simulink model "ElectricVehicleThermalManagementWithHeatPump"  (R2024b)
settings: Solver=VariableStepAuto  StartTime=0.0  StopTime=3600  RelTol=1e-3  AbsTol=1e-3
PreLoadFcn:
  | init_nmpc
InitFcn:
  | init_nmpc
model workspace: external: MATLAB File ElectricVehicleThermalManagementWithHeatPumpParameters.m (data not in the file)
values from neighbouring files (symbols this model uses):
  battery_C1_LUT = [1913.6 12447 30609 ... (first row only)    [ElectricVehicleThermalManagementWithHeatPumpParameters.m]
  battery_capacity_LUT = [280.081 276.25 276.392]    [ElectricVehicleThermalManagementWithHeatPumpParameters.m]
  battery_cell_cp = 795    [ElectricVehicleThermalManagementWithHeatPumpParameters.m]
  battery_cell_mass = 2.5    [ElectricVehicleThermalManagementWithHeatPumpParameters.m]
  battery_Em_LUT = [3.4966 3.5057 3.5148 ... (first row only)    [ElectricVehicleThermalManagementWithHeatPumpParameters.m]
  battery_N_cells = 20    [ElectricVehicleThermalManagementWithHeatPumpParameters.m]
  battery_Qe_init = 0    [ElectricVehicleThermalManagementWithHeatPumpParameters.m]
  battery_R0_LUT = [0.0117 0.0085 0.009 ... (first row only)    [ElectricVehicleThermalManagementWithHeatPumpParameters.m]
  battery_R1_LUT = [0.0109 0.0029 0.0013 ... (first row only)    [ElectricVehicleThermalManagementWithHeatPumpParameters.m]
  battery_SOC_LUT = [0; 0.1; 0.25; 0.5; 0.75; 0.9; 1]    [ElectricVehicleThermalManagementWithHeatPumpParameters.m]
  battery_T_init = -10    [ElectricVehicleThermalManagementWithHeatPumpParameters.m]
  battery_temperature_LUT = [5 20 40]    [ElectricVehicleThermalManagementWithHeatPumpParameters.m]
  cabin_duct_area = 0.04    [ElectricVehicleThermalManagementWithHeatPumpParameters.m]
  cabin_T_init = -10    [ElectricVehicleThermalManagementWithHeatPumpParameters.m]
  chiller_area_primary = 0.43982297150257105    (= 0.439822971503)    [ElectricVehicleThermalManagementWithHeatPumpParameters.m]
  chiller_N_baffles = 3    [ElectricVehicleThermalManagementWithHeatPumpParameters.m]
  chiller_N_tubes = 100    [ElectricVehicleThermalManagementWithHeatPumpParameters.m]
  chiller_tube_D = 0.0035    [ElectricVehicleThermalManagementWithHeatPumpParameters.m]
  chiller_tube_L = 0.4    [ElectricVehicleThermalManagementWithHeatPumpParameters.m]
  chiller_wall_conductivity = 240    [ElectricVehicleThermalManagementWithHeatPumpParameters.m]
  chiller_wall_thickness = 0.0001    [ElectricVehicleThermalManagementWithHeatPumpParameters.m]
  cond_evap_air_area_flow = 0.3906    [ElectricVehicleThermalManagementWithHeatPumpParameters.m]
  cond_evap_air_area_primary = 1.4834999999999998    (= 1.4835)    [ElectricVehicleThermalManagementWithHeatPumpParameters.m]
  cond_evap_W = 0.015    [ElectricVehicleThermalManagementWithHeatPumpParameters.m]
  cond_evap_wall_conductivity = 240    [ElectricVehicleThermalManagementWithHeatPumpParameters.m]
  cond_evap_wall_thickness = 0.0001    [ElectricVehicleThermalManagementWithHeatPumpParameters.m]
  coolant_channel_D = 0.0092    [ElectricVehicleThermalManagementWithHeatPumpParameters.m]
  coolant_pipe_D = 0.019    [ElectricVehicleThermalManagementWithHeatPumpParameters.m]
  coolant_T_init = -10    [ElectricVehicleThermalManagementWithHeatPumpParameters.m]
  coolant_tank_area = 0.0121    [ElectricVehicleThermalManagementWithHeatPumpParameters.m]
  coolant_tank_volume = 1.25    [ElectricVehicleThermalManagementWithHeatPumpParameters.m]
  coolant_valve_D_ratio_max = 0.95    [ElectricVehicleThermalManagementWithHeatPumpParameters.m]
  coolant_valve_D_ratio_min = 0.001    [ElectricVehicleThermalManagementWithHeatPumpParameters.m]
  coolant_valve_displacement = 0.0063    [ElectricVehicleThermalManagementWithHeatPumpParameters.m]
  coolant_valve_S_max = 0.0053    [ElectricVehicleThermalManagementWithHeatPumpParameters.m]
  evaporator_air_area_flow = 0.12    [ElectricVehicleThermalManagementWithHeatPumpParameters.m]
  evaporator_air_area_primary = 0.4323    [ElectricVehicleThermalManagementWithHeatPumpParameters.m]
  evaporator_W = 0.015    [ElectricVehicleThermalManagementWithHeatPumpParameters.m]
  evaporator_wall_conductivity = 240    [ElectricVehicleThermalManagementWithHeatPumpParameters.m]
  evaporator_wall_thickness = 0.0001    [ElectricVehicleThermalManagementWithHeatPumpParameters.m]
  expansion_valve_D_ratio_max = 0.9    [ElectricVehicleThermalManagementWithHeatPumpParameters.m]
  hex_area_primary = 0.070371675440411369    (= 0.0703716754404)    [ElectricVehicleThermalManagementWithHeatPumpParameters.m]
  hex_N_tubes = 64    [ElectricVehicleThermalManagementWithHeatPumpParameters.m]
  hex_tube_D = 0.0035    [ElectricVehicleThermalManagementWithHeatPumpParameters.m]
  hex_wall_conductivity = 240    [ElectricVehicleThermalManagementWithHeatPumpParameters.m]
  hex_wall_thickness = 0.0001    [ElectricVehicleThermalManagementWithHeatPumpParameters.m]
  inner_cond_air_area_flow = 0.1953    [ElectricVehicleThermalManagementWithHeatPumpParameters.m]
  inner_cond_air_area_primary = 0.99520000000000008    (= 0.9952)    [ElectricVehicleThermalManagementWithHeatPumpParameters.m]
  inner_cond_W = 0.02    [ElectricVehicleThermalManagementWithHeatPumpParameters.m]
  inner_cond_wall_conductivity = 240    [ElectricVehicleThermalManagementWithHeatPumpParameters.m]
  inner_cond_wall_thickness = 0.0001    [ElectricVehicleThermalManagementWithHeatPumpParameters.m]
  pump_speed_max = 1000    [ElectricVehicleThermalManagementWithHeatPumpParameters.m]
  radiator_air_area_flow = 0.097499999999999989    (= 0.0975)    [ElectricVehicleThermalManagementWithHeatPumpParameters.m]
  radiator_air_area_primary = 0.43687499999999996    (= 0.436875)    [ElectricVehicleThermalManagementWithHeatPumpParameters.m]
  radiator_W = 0.015    [ElectricVehicleThermalManagementWithHeatPumpParameters.m]
  radiator_wall_conductivity = 240    [ElectricVehicleThermalManagementWithHeatPumpParameters.m]
  radiator_wall_thickness = 0.0001    [ElectricVehicleThermalManagementWithHeatPumpParameters.m]
  refrigerant_p_init = 0.2    [ElectricVehicleThermalManagementWithHeatPumpParameters.m]
  refrigerant_pipe_D = 0.01    [ElectricVehicleThermalManagementWithHeatPumpParameters.m]
  refrigerant_valve_D_ratio_max = 0.95    [ElectricVehicleThermalManagementWithHeatPumpParameters.m]
  refrigerant_valve_displacement = 0.005    [ElectricVehicleThermalManagementWithHeatPumpParameters.m]
libraries: fl_lib x227, nesl_utility x162, SimscapeFluids_lib x30, LiBatteryElements_lib x16, slpidlib x3, SignalEditorBlockLib x1
(part 5 of 13)

== system ElectricVehicleThermalManagementWithHeatPump/Evaporator ==
  Evaporator : SimscapeFluids_lib/Heat Exchangers/Two-Phase Fluid - Moist Air/Condenser Evaporator (2P-MA)  flow_arrangement=fluids.heat_exchangers.enum.FlowArrangement2PMA.Cross  cross_flow_arrangement=fluids.heat_exchangers.enum.CrossFlowArrangement2PMA.UnmixedUnmixed  R_wall=evaporator_wall_thickness / evaporator_air_area_primary / evaporator_wall_conductivity K/W  area_A1=pi * refrigerant_pipe_D^2 / 4 m^2  area_B1=pi * refrigerant_pipe_D^2 / 4 m^2  area_A2=cabin_duct_area m^2  area_B2=cabin_duct_area m^2  tube_num_2P=evaporator_N_tubes  tube_length_2P=evaporator_L m  tube_cross_section_2P=fluids.heat_exchangers.enum.TubeCrossSection.Rectangular  tube_diameter_2P=0.1 m  tube_width_2P=evaporator_W m  tube_height_2P=evaporator_tube_H m  tube_inner_diameter_2P=0.05 m  tube_outer_diameter_2P=0.1 m  tube_flow_area_2P=0.01 m^2  tube_wetted_perimeter_2P=0.4 m  tube_heat_perimeter_2P=0.4 m  tube_pressure_loss_spec_2P=fluids.heat_exchangers.enum.TubePressureLossSpec2P.Haaland  tube_loss_coeff_2P=10  tube_local_pressure_loss_spec_2P=fluids.heat_exchangers.enum.LocalLossSpec.AggregateLength  tube_length_add_2P=evaporator_tube_Leq m  tube_local_loss_coefficient_2P=0.1  tube_roughness_pressure_2P=15e-6 m  tube_Re_lam_pressure_2P=2000  tube_Re_tur_pressure_2P=4000  tube_shape_factor_generic_2P=64  tube_heat_coeff_spec_2P=fluids.heat_exchangers.enum.TubeHeatCoeffSpec2P.GneilinskiCavalliniZecchin  tube_colburn_coeff_liq_2P=[.023, .8, .33]  tube_colburn_coeff_mix_2P=[.05, .8, .33]  tube_colburn_coeff_vap_2P=[.023, .8, .33]  tube_roughness_heat_2P=15e-6 m  tube_Re_lam_heat_2P=2000  tube_Re_tur_heat_2P=4000  tube_Nu_lam_generic_2P=3.66  fouling_factor_2P=0.1 m^2*K/kW  fin_area_2P=evaporator_tube_area_webs m^2  fin_efficiency_2P=0.6  energy_spec_2P=foundation.enum.energy_spec.void_fraction  p_init_2P=refrigerant_p_init MPa  T_init_2P=293.15 K  x_init_2P=0.5  alpha_init_2P=refrigerant_alpha_init  h_init_2P=1500 kJ/kg  u_init_2P=1500 kJ/kg  flow_geometry_MA=fluids.heat_exchangers.enum.FlowGeometryMA.Generic  tube_num_MA=1  tube_length_MA=5 m  tube_cross_section_MA=fluids.heat_exchangers.enum.TubeCrossSection.Circular  tube_diameter_MA=0.1 m  tube_width_MA=0.1 m  tube_height_MA=0.1 m  tube_inner_diameter_MA=0.05 m  tube_outer_diameter_MA=0.1 m  tube_flow_area_MA=0.01 m^2  tube_wetted_perimeter_MA=0.4 m  tube_heat_perimeter_MA=0.4 m  tube_pressure_loss_spec_MA=fluids.heat_exchangers.enum.TubePressureLossSpec.Haaland  tube_loss_coeff_MA=10  tube_local_pressure_loss_spec_MA=fluids.heat_exchangers.enum.LocalLossSpec.AggregateLength  tube_length_add_MA=0.1 m  tube_local_loss_coefficient_MA=0.1  tube_roughness_pressure_MA=15e-6 m  tube_Re_lam_pressure_MA=2000  tube_Re_tur_pressure_MA=4000  tube_shape_factor_generic_MA=64  tube_heat_coeff_spec_MA=fluids.heat_exchangers.enum.TubeHeatCoeffSpec.Gneilinski  tube_colburn_coeff_MA=[.023, .8, .33]  tube_roughness_heat_MA=15e-6 m  tube_Re_lam_heat_MA=2000  tube_Re_tur_heat_MA=4000  tube_Nu_lam_generic_MA=3.66  bank_arrangement_MA=fluids.heat_exchangers.enum.BankArrangement.Inline  bank_num_rows_MA=5  bank_tubes_per_row_MA=5  bank_width_MA=1 m  bank_tube_diameter_MA=0.05 m  bank_longitudinal_pitch_MA=0.15 m  bank_transverse_pitch_MA=0.15 m  bank_pressure_loss_spec_MA=fluids.heat_exchangers.enum.BankPressureLossSpec.Martin  bank_euler_MA=10  bank_heat_coeff_spec_MA=fluids.heat_exchangers.enum.BankHeatCoeffSpec.Martin  bank_colburn_coeff_MA=[.27, .63, .36]  generic_flow_area_MA=evaporator_air_area_flow m^2  generic_heat_area_MA=evaporator_air_area_primary m^2  generic_volume_MA=evaporator_air_area_flow * evaporator_W m^3  generic_loss_coeff_MA=10  generic_colburn_coeff_MA=[0.27, 0.63, 0.36]  fouling_factor_MA=0.1 m^2*K/kW  fin_area_MA=evaporator_air_area_fins m^2  fin_efficiency_MA=0.7  p_init_MA=cabin_p_init MPa  T_init_MA=cabin_T_init degC  humidity_spec_MA=foundation.enum.HumiditySpec.RelativeHumidity  RH_init_MA=cabin_RH_init  x_w_init_MA=0.01  y_w_init_MA=0.01  HR_init_MA=0.01  Tw_init_MA=287 K  trace_gas_spec_MA=foundation.enum.trace_gas_spec.mole_fraction  x_g_init_MA=0.001  y_g_init_MA=cabin_CO2_init  r_d_init_MA=0  RH_ws_MA=1  time_constant_cond_MA=1e-3 s  time_constant_evap_MA=1e-3 s  fraction_entrained_MA=1
      settings: InternalSimscapePortConfiguration="{\"Bottom\":[],\"Left\":[{\"id\":\"A1\",\"label\":\"A1\",\"type\":\"foundation.two_phase_fluid.two_phase_fluid\"},{\"id\":\"Z\",\"label\":\"Z\",\"type\":\"output\"},{\"id\":\"B1\",\"label\":\"B1\",\"type\":\"foundation.two_phase_fluid.two_phase_fluid\"}],\"Right\":[{\"id\":\"A2\",\"label\":\"A2\",\"type\":\"foundation.moist_air.moist_air\"},{\"id\":\"W\",\"label\":\"W\",\"type\":\"output\"},{\"id\":\"B2\",\"label\":\"B2\",\"type\":\"foundation.moist_air.moist_air\"}],\"Top\":[]}"
  Flow Resistance (2P) : fl_lib/Two-Phase Fluid/Elements/Flow Resistance (2P)  delta_p_nominal=1e-4 MPa  mdot_nominal=0.01 kg/s  v_nominal=0 m^3/kg  area=pi * refrigerant_pipe_D^2 / 4 m^2  laminar_fraction=1e-3
      settings: InternalSimscapePortConfiguration="{\"Bottom\":[],\"Left\":[{\"id\":\"A\",\"label\":\"A\",\"type\":\"foundation.two_phase_fluid.two_phase_fluid\"}],\"Right\":[{\"id\":\"B\",\"label\":\"B\",\"type\":\"foundation.two_phase_fluid.two_phase_fluid\"}],\"Top\":[]}"
  PS-Simulink Converter{,1..3} (4 alike) : nesl_utility/PS-Simulink Converter  PhysicalDomain=network_engine_domain  SubClassName=ps_output  LeftPortType=input  RightPortType=output  PseudoPeriodic=off  Frequencies=[]  VectorFormat=inherit  Unit=inherit  AffineConversion=off
  Pressure & Temperature Sensor (MA) : fl_lib/Moist Air/Sensors/Pressure & Temperature Sensor (MA)  reference=foundation.enum.MeasurementReference.absolute  pressure=true  pressure_spec=foundation.enum.PressureMeasementSpec.Absolute  temperature=true
      settings: InternalSimscapePortConfiguration="{\"Bottom\":[{\"id\":\"T\",\"label\":\"T\",\"type\":\"output\"}],\"Left\":[{\"id\":\"A\",\"label\":\"A\",\"type\":\"foundation.moist_air.moist_air\"}],\"Right\":[{\"id\":\"Pa\",\"label\":\"Pa\",\"type\":\"output\"}],\"Top\":[]}"
  Pressure & Temperature Sensor (MA)1 : fl_lib/Moist Air/Sensors/Pressure & Temperature Sensor (MA)  reference=foundation.enum.MeasurementReference.absolute  pressure=true  pressure_spec=foundation.enum.PressureMeasementSpec.Absolute  temperature=true
      settings: InternalSimscapePortConfiguration="{\"Bottom\":[{\"id\":\"T\",\"label\":\"T\",\"type\":\"output\"}],\"Left\":[{\"id\":\"A\",\"label\":\"A\",\"type\":\"foundation.moist_air.moist_air\"}],\"Right\":[{\"id\":\"Pa\",\"label\":\"Pa\",\"type\":\"output\"}],\"Top\":[]}"
  SR7 : Subsystem
  SR8 : Subsystem
  Scope : Scope
  To Workspace : ToWorkspace  VariableName=airEvapPressure_out  SampleTime=-1
  To Workspace1 : ToWorkspace  VariableName=airEvapTemp_out  SampleTime=-1
  To Workspace2 : ToWorkspace  VariableName=airEvapPressure_in  SampleTime=-1
  To Workspace3 : ToWorkspace  VariableName=airEvapTemp_in  SampleTime=-1
  A : PMIOPort  Side=Left
  D : PMIOPort  Port=2  Side=Left
  B : PMIOPort  Port=3  Side=Right
  C : PMIOPort  Port=4  Side=Right
  wires:
  PS-Simulink Converter/1 -> To Workspace/1
  PS-Simulink Converter3/1 -> Scope/1, To Workspace1/1
  PS-Simulink Converter1/1 -> To Workspace2/1
  PS-Simulink Converter2/1 -> To Workspace3/1
  connections:
  SR8/LConn1 -- Evaporator/LConn3
  SR7/RConn1 -- Evaporator/LConn1
  SR8/RConn1 -- Flow Resistance (2P)/LConn1
  Evaporator/RConn3 -- Pressure & Temperature Sensor (MA)1/LConn1 -- C/RConn1
  Flow Resistance (2P)/RConn1 -- B/RConn1
  Evaporator/RConn1 -- D/RConn1 -- Pressure & Temperature Sensor (MA)/LConn1
  SR7/LConn1 -- A/RConn1
  PS-Simulink Converter/LConn1 -- Pressure & Temperature Sensor (MA)/RConn1
  PS-Simulink Converter1/LConn1 -- Pressure & Temperature Sensor (MA)1/RConn1
  PS-Simulink Converter2/LConn1 -- Pressure & Temperature Sensor (MA)1/RConn2
  PS-Simulink Converter3/LConn1 -- Pressure & Temperature Sensor (MA)/RConn2

== system ElectricVehicleThermalManagementWithHeatPump/Evaporator Expansion Valve ==
  Evaporator Expansion Valve : SimscapeFluids_lib/Two-Phase Fluid/Valves & Orifices/Orifice (2P)  orifice_type=foundation.enum.constant_variable.variable  constant_liquid_orifice_parameterization=fluids.two_phase_fluid.valves_orifices.enum.LiquidConstantOrificeParameterization.Area  variable_liquid_orifice_parameterization=fluids.two_phase_fluid.valves_orifices.enum.LiquidOrificeParameterization.LinearArea  mdot_nominal_constant=0.1 kg/s  delta_p_nominal_constant=0.001 MPa  orifice_area_constant=1e-4 m^2  S_min=0 m  del_S=refrigerant_valve_displacement m  open_orientation=fluids.two_phase_fluid.valves_orifices.enum.OrificeOrientation.Positive  mdot_nominal_max=0.1 kg/s  delta_p_nominal_max=0.001 MPa  orifice_area_max=pi * (expansion_valve_D_ratio_max*refrigerant_pipe_D)^2 / 4 m^2  S_TLU=[0, .002, .004, .007, .017] m  orifice_area_TLU=[1e-10, 2e-05, 4e-05, 6e-05, 8e-05, .0001] m^2  energy_spec=foundation.enum.energy_spec.temperature  p_inlet=0.101325 MPa  T_inlet=293.15 K  x_inlet=0  alpha_inlet=0  h_inlet=400 kJ/kg  u_inlet=400 kJ/kg  Cd=0.7  pressure_recovery=true  leakage_fraction=1e-6  smoothing_factor=0.01  B_lam=0.999  tau_x=0.1 s  area=pi * refrigerant_pipe_D^2 / 4 m^2  vapor_orifice_parameterization=fluids.two_phase_fluid.valves_orifices.enum.VaporOrificeParameterization.Cv  opening_characteristic=fluids.two_phase_fluid.valves_orifices.enum.OpeningCharacteristics.Linear  Cv_constant=4  Cv_max=4  S_Cv_TLU=[0, .003, .006, .009, .012, .015] m  Cv_TLU=[1e-06, .8, 1.6, 2.4, 3.2, 4]  xT_Cv=0.7  Kv_constant=3.6  Kv_max=3.6  S_Kv_TLU=[0, .003, .006, .009, .012, .015] m  Kv_TLU=[1e-06, .72, 1.44, 2.16, 2.88, 3.6]  xT_Kv=0.7  S_orifice_area_TLU=[0, .003, .006, .009, .012, .015] m
      settings: InternalSimscapePortConfiguration="{\"Bottom\":[],\"Left\":[{\"id\":\"A\",\"label\":\"A\",\"type\":\"foundation.two_phase_fluid.two_phase_fluid\"},{\"id\":\"S\",\"label\":\"S\",\"type\":\"input\"}],\"Right\":[{\"id\":\"B\",\"label\":\"B\",\"type\":\"foundation.two_phase_fluid.two_phase_fluid\"}],\"Top\":[]}"
  Max Valve Displacement [m] : Gain  Gain=refrigerant_valve_displacement
  Simulink-PS Converter : nesl_utility/Simulink-PS Converter  PhysicalDomain=network_engine_domain  SubClassName=ps_input  LeftPortType=input  RightPortType=output  PseudoPeriodic=off  Frequencies=[]  NoiseDistribution=none  NoiseParameters=[]  Unit=m  AffineConversion=off  FilteringAndDerivatives=provide  SimscapeFilterOrder=1  InputFilterTimeConstant=0.001  UdotUserProvided=0
  Transfer Fcn : TransferFcn  Denominator=[1 1]
  A : PMIOPort  Side=Left
  B : PMIOPort  Port=2  Side=Right
  wires:
  Transfer Fcn/1 -> Max Valve Displacement [m]/1
  [cmd_exv_evap] -> Transfer Fcn/1
  Max Valve Displacement [m]/1 -> Simulink-PS Converter/1
  connections:
  Evaporator Expansion Valve/LConn2 -- Simulink-PS Converter/RConn1
  Evaporator Expansion Valve/LConn1 -- A/RConn1
  Evaporator Expansion Valve/RConn1 -- B/RConn1

== system ElectricVehicleThermalManagementWithHeatPump/Heat Exchanger ==
  Flow Rate Sensor (TL) : fl_lib/Thermal Liquid/Sensors/Flow Rate Sensor (TL)  mass_flow_measure=true  volumetric_flow_measure=false  energy_flow_measure=true
      settings: InternalSimscapePortConfiguration="{\"Bottom\":[{\"id\":\"PHI\",\"label\":\"φ\",\"type\":\"output\"}],\"Left\":[{\"id\":\"A\",\"label\":\"A\",\"type\":\"foundation.thermal_liquid.thermal_liquid\"}],\"Right\":[{\"id\":\"B\",\"label\":\"B\",\"type\":\"foundation.thermal_liquid.thermal_liquid\"},{\"id\":\"M\",\"label\":\"M\",\"type\":\"output\"}],\"Top\":[]}"
  Heat Exchanger : SimscapeFluids_lib/Heat Exchangers/Two-Phase Fluid - Thermal Liquid/Condenser Evaporator (TL-2P)  flow_arrangement=fluids.heat_exchangers.enum.FlowArrangementTL2P.Cross  cross_flow_arrangement=fluids.heat_exchangers.enum.CrossFlowArrangementTL2P.UnmixedMixed  R_wall=hex_wall_thickness / hex_area_primary / hex_wall_conductivity K/W  area_A1=pi * coolant_pipe_D^2 / 4 m^2  area_B1=pi * coolant_pipe_D^2 / 4 m^2  area_A2=pi * refrigerant_pipe_D^2 / 4 m^2  area_B2=pi * refrigerant_pipe_D^2 / 4 m^2  flow_geometry_TL=fluids.heat_exchangers.enum.FlowGeometryTL.AcrossTubeBank  tube_num_TL=1  tube_length_TL=5 m  tube_cross_section_TL=fluids.heat_exchangers.enum.TubeCrossSection.Circular  tube_diameter_TL=0.1 m  tube_width_TL=0.1 m  tube_height_TL=0.1 m  tube_inner_diameter_TL=0.05 m  tube_outer_diameter_TL=0.1 m  tube_flow_area_TL=0.01 m^2  tube_wetted_perimeter_TL=0.4 m  tube_heat_perimeter_TL=0.4 m  tube_pressure_loss_spec_TL=fluids.heat_exchangers.enum.TubePressureLossSpec.Haaland  tube_loss_coeff_TL=10  tube_local_pressure_loss_spec_TL=fluids.heat_exchangers.enum.LocalLossSpec.AggregateLength  tube_length_add_TL=0.1 m  tube_local_loss_coefficient_TL=0.1  tube_roughness_pressure_TL=15e-6 m  tube_Re_lam_pressure_TL=2000  tube_Re_tur_pressure_TL=4000  tube_shape_factor_generic_TL=64  tube_heat_coeff_spec_TL=fluids.heat_exchangers.enum.TubeHeatCoeffSpec.Gneilinski  tube_colburn_coeff_TL=[.023, .8, .33]  tube_roughness_heat_TL=15e-6 m  tube_Re_lam_heat_TL=2000  tube_Re_tur_heat_TL=4000  tube_Nu_lam_generic_TL=3.66  bank_arrangement_TL=fluids.heat_exchangers.enum.BankArrangement.Staggered  bank_num_rows_TL=sqrt(hex_N_tubes)  bank_tubes_per_row_TL=sqrt(hex_N_tubes)  bank_width_TL=hex_tube_L m  bank_tube_diameter_TL=hex_tube_D m  bank_longitudinal_pitch_TL=2 * hex_tube_D m  bank_transverse_pitch_TL=2 * hex_tube_D m  bank_pressure_loss_spec_TL=fluids.heat_exchangers.enum.BankPressureLossSpec.Martin  bank_euler_TL=10  bank_heat_coeff_spec_TL=fluids.heat_exchangers.enum.BankHeatCoeffSpec.Martin  bank_colburn_coeff_TL=[.27, .63, .36]  generic_flow_area_TL=0.01 m^2  generic_heat_area_TL=2 m^2  generic_volume_TL=0.05 m^3  generic_loss_coeff_TL=10  generic_colburn_coeff_TL=[.023, .8, .33]  fouling_factor_TL=0.1 m^2*K/kW  fin_area_TL=0 m^2  fin_efficiency_TL=0  p_init_TL=coolant_p_init MPa  T_init_TL=coolant_T_init degC  tube_num_2P=hex_N_tubes  tube_length_2P=hex_tube_L m  tube_cross_section_2P=fluids.heat_exchangers.enum.TubeCrossSection.Circular  tube_diameter_2P=hex_tube_D m  tube_width_2P=0.1 m  tube_height_2P=0.1 m  tube_inner_diameter_2P=0.05 m  tube_outer_diameter_2P=0.1 m  tube_flow_area_2P=0.01 m^2  tube_wetted_perimeter_2P=0.4 m  tube_heat_perimeter_2P=0.4 m  tube_pressure_loss_spec_2P=fluids.heat_exchangers.enum.TubePressureLossSpec2P.Haaland  tube_loss_coeff_2P=10  tube_local_pressure_loss_spec_2P=fluids.heat_exchangers.enum.LocalLossSpec.AggregateLength  tube_length_add_2P=hex_tube_Leq m  tube_local_loss_coefficient_2P=0.1  tube_roughness_pressure_2P=15e-6 m  tube_Re_lam_pressure_2P=2000  tube_Re_tur_pressure_2P=4000  tube_shape_factor_generic_2P=64  tube_heat_coeff_spec_2P=fluids.heat_exchangers.enum.TubeHeatCoeffSpec2P.GneilinskiCavalliniZecchin  tube_colburn_coeff_liq_2P=[.023, .8, .33]  tube_colburn_coeff_mix_2P=[.05, .8, .33]  tube_colburn_coeff_vap_2P=[.023, .8, .33]  tube_roughness_heat_2P=15e-6 m  tube_Re_lam_heat_2P=2000  tube_Re_tur_heat_2P=4000  tube_Nu_lam_generic_2P=3.66  fouling_factor_2P=0.1 m^2*K/kW  fin_area_2P=0 m^2  fin_efficiency_2P=0  energy_spec_2P=foundation.enum.energy_spec.void_fraction  p_init_2P=refrigerant_p_init MPa  T_init_2P=293.15 K  x_init_2P=0.5  alpha_init_2P=refrigerant_alpha_init  h_init_2P=1500 kJ/kg  u_init_2P=1500 kJ/kg
      settings: InternalSimscapePortConfiguration="{\"Bottom\":[],\"Left\":[{\"id\":\"A1\",\"label\":\"A1\",\"type\":\"foundation.thermal_liquid.thermal_liquid\"},{\"id\":\"B1\",\"label\":\"B1\",\"type\":\"foundation.thermal_liquid.thermal_liquid\"}],\"Right\":[{\"id\":\"A2\",\"label\":\"A2\",\"type\":\"foundation.two_phase_fluid.two_phase_fluid\"},{\"id\":\"B2\",\"label\":\"B2\",\"type\":\"foundation.two_phase_fluid.two_phase_fluid\"}],\"Top\":[{\"id\":\"Z\",\"label\":\"Z\",\"type\":\"output\"}]}"
  PS-Simulink Converter : nesl_utility/PS-Simulink Converter  PhysicalDomain=network_engine_domain  SubClassName=ps_output  LeftPortType=input  RightPortType=output  PseudoPeriodic=off  Frequencies=[]  VectorFormat=inherit  Unit=inherit  AffineConversion=off
  PS-Simulink Converter1 : nesl_utility/PS-Simulink Converter  PhysicalDomain=network_engine_domain  SubClassName=ps_output  LeftPortType=input  RightPortType=output  PseudoPeriodic=off  Frequencies=[]  VectorFormat=inherit  Unit=inherit  AffineConversion=off
  PS-Simulink Converter2 : nesl_utility/PS-Simulink Converter  PhysicalDomain=network_engine_domain  SubClassName=ps_output  LeftPortType=input  RightPortType=output  PseudoPeriodic=off  Frequencies=[]  VectorFormat=inherit  Unit=inherit  AffineConversion=off
  Pressure & Temperature Sensor (TL) : fl_lib/Thermal Liquid/Sensors/Pressure & Temperature Sensor (TL)  reference=foundation.enum.MeasurementReference.absolute  pressure=false  pressure_spec=foundation.enum.PressureMeasementSpec.Absolute  temperature=true
      settings: InternalSimscapePortConfiguration="{\"Bottom\":[{\"id\":\"T\",\"label\":\"T\",\"type\":\"output\"}],\"Left\":[{\"id\":\"A\",\"label\":\"A\",\"type\":\"foundation.thermal_liquid.thermal_liquid\"}],\"Right\":[],\"Top\":[]}"
  Pressure & Temperature Sensor (TL)1 : fl_lib/Thermal Liquid/Sensors/Pressure & Temperature Sensor (TL)  reference=foundation.enum.MeasurementReference.absolute  pressure=false  pressure_spec=foundation.enum.PressureMeasementSpec.Absolute  temperature=true
      settings: InternalSimscapePortConfiguration="{\"Bottom\":[{\"id\":\"T\",\"label\":\"T\",\"type\":\"output\"}],\"Left\":[{\"id\":\"A\",\"label\":\"A\",\"type\":\"foundation.thermal_liquid.thermal_liquid\"}],\"Right\":[],\"Top\":[]}"
  SR5 : Subsystem
  SR6 : Subsystem
  Scope : Scope
  Scope1 : Scope
  Scope2 : Scope
  To Workspace : ToWorkspace  VariableName=heatExchangerCoolantT_outK  SampleTime=-1
  To Workspace1 : ToWorkspace  VariableName=heatExchangerCoolantT_inK  SampleTime=-1
  To Workspace2 : ToWorkspace  VariableName=mf_htxClnt  SampleTime=-1
  D : PMIOPort  Side=Left
  A : PMIOPort  Port=2  Side=Left
  C : PMIOPort  Port=3  Side=Right
  B : PMIOPort  Port=4  Side=Right
  wires:
  PS-Simulink Converter/1 -> To Workspace/1, Scope/1
  PS-Simulink Converter1/1 -> Scope1/1, To Workspace1/1
  PS-Simulink Converter2/1 -> To Workspace2/1, Scope2/1
  connections:
  Heat Exchanger/RConn2 -- SR6/LConn1
  SR6/RConn1 -- B/RConn1
  Heat Exchanger/RConn1 -- SR5/RConn1
  SR5/LConn1 -- A/RConn1
  C/RConn1 -- Pressure & Temperature Sensor (TL)1/LConn1 -- Heat Exchanger/LConn2
  Pressure & Temperature Sensor (TL)/LConn1 -- D/RConn1 -- Flow Rate Sensor (TL)/RConn1
  PS-Simulink Converter/LConn1 -- Pressure & Temperature Sensor (TL)/RConn1
  PS-Simulink Converter1/LConn1 -- Pressure & Temperature Sensor (TL)1/RConn1
  PS-Simulink Converter2/LConn1 -- Flow Rate Sensor (TL)/RConn2
  Flow Rate Sensor (TL)/LConn1 -- Heat Exchanger/LConn1

== system ElectricVehicleThermalManagementWithHeatPump/Heat Pump Expansion Valve ==
  Heat Pump Expansion Valve : SimscapeFluids_lib/Two-Phase Fluid/Valves & Orifices/Orifice (2P)  orifice_type=foundation.enum.constant_variable.variable  constant_liquid_orifice_parameterization=fluids.two_phase_fluid.valves_orifices.enum.LiquidConstantOrificeParameterization.Area  variable_liquid_orifice_parameterization=fluids.two_phase_fluid.valves_orifices.enum.LiquidOrificeParameterization.LinearArea  mdot_nominal_constant=0.1 kg/s  delta_p_nominal_constant=0.001 MPa  orifice_area_constant=1e-4 m^2  S_min=0 m  del_S=refrigerant_valve_displacement m  open_orientation=fluids.two_phase_fluid.valves_orifices.enum.OrificeOrientation.Positive  mdot_nominal_max=0.1 kg/s  delta_p_nominal_max=0.001 MPa  orifice_area_max=pi * (expansion_valve_D_ratio_max*refrigerant_pipe_D)^2 / 4 m^2  S_TLU=[0, .002, .004, .007, .017] m  orifice_area_TLU=[1e-10, 2e-05, 4e-05, 6e-05, 8e-05, .0001] m^2  energy_spec=foundation.enum.energy_spec.temperature  p_inlet=0.101325 MPa  T_inlet=293.15 K  x_inlet=0  alpha_inlet=0  h_inlet=400 kJ/kg  u_inlet=400 kJ/kg  Cd=0.7  pressure_recovery=true  leakage_fraction=1e-6  smoothing_factor=0.01  B_lam=0.999  tau_x=0.1 s  area=pi * refrigerant_pipe_D^2 / 4 m^2  vapor_orifice_parameterization=fluids.two_phase_fluid.valves_orifices.enum.VaporOrificeParameterization.Cv  opening_characteristic=fluids.two_phase_fluid.valves_orifices.enum.OpeningCharacteristics.Linear  Cv_constant=4  Cv_max=4  S_Cv_TLU=[0, .003, .006, .009, .012, .015] m  Cv_TLU=[1e-06, .8, 1.6, 2.4, 3.2, 4]  xT_Cv=0.7  Kv_constant=3.6  Kv_max=3.6  S_Kv_TLU=[0, .003, .006, .009, .012, .015] m  Kv_TLU=[1e-06, .72, 1.44, 2.16, 2.88, 3.6]  xT_Kv=0.7  S_orifice_area_TLU=[0, .003, .006, .009, .012, .015] m
      settings: InternalSimscapePortConfiguration="{\"Bottom\":[],\"Left\":[{\"id\":\"A\",\"label\":\"A\",\"type\":\"foundation.two_phase_fluid.two_phase_fluid\"},{\"id\":\"S\",\"label\":\"S\",\"type\":\"input\"}],\"Right\":[{\"id\":\"B\",\"label\":\"B\",\"type\":\"foundation.two_phase_fluid.two_phase_fluid\"}],\"Top\":[]}"
  Max Valve Displacement [m] : Gain  Gain=refrigerant_valve_displacement
  PS-Simulink Converter : nesl_utility/PS-Simulink Converter  PhysicalDomain=network_engine_domain  SubClassName=ps_output  LeftPortType=input  RightPortType=output  PseudoPeriodic=off  Frequencies=[]  VectorFormat=inherit  Unit=inherit  AffineConversion=off
  PS-Simulink Converter1 : nesl_utility/PS-Simulink Converter  PhysicalDomain=network_engine_domain  SubClassName=ps_output  LeftPortType=input  RightPortType=output  PseudoPeriodic=off  Frequencies=[]  VectorFormat=inherit  Unit=inherit  AffineConversion=off
  "Pressure, Temperature & Internal Energy Sensor (2P)" : fl_lib/Two-Phase Fluid/Sensors/Pressure, Temperature & Internal Energy Sensor (2P)  reference=foundation.enum.MeasurementReference.absolute  pressure=true  pressure_spec=foundation.enum.PressureMeasementSpec.Absolute  temperature=false  internal_energy=false
      settings: InternalSimscapePortConfiguration="{\"Bottom\":[],\"Left\":[{\"id\":\"A\",\"label\":\"A\",\"type\":\"foundation.two_phase_fluid.two_phase_fluid\"}],\"Right\":[{\"id\":\"Pa\",\"label\":\"Pa\",\"type\":\"output\"}],\"Top\":[]}"
  "Pressure, Temperature & Internal Energy Sensor (2P)1" : fl_lib/Two-Phase Fluid/Sensors/Pressure, Temperature & Internal Energy Sensor (2P)  reference=foundation.enum.MeasurementReference.absolute  pressure=true  pressure_spec=foundation.enum.PressureMeasementSpec.Absolute  temperature=false  internal_energy=false
      settings: InternalSimscapePortConfiguration="{\"Bottom\":[],\"Left\":[{\"id\":\"A\",\"label\":\"A\",\"type\":\"foundation.two_phase_fluid.two_phase_fluid\"}],\"Right\":[{\"id\":\"Pa\",\"label\":\"Pa\",\"type\":\"output\"}],\"Top\":[]}"
  Scope : Scope
  Simulink-PS Converter : nesl_utility/Simulink-PS Converter  PhysicalDomain=network_engine_domain  SubClassName=ps_input  LeftPortType=input  RightPortType=output  PseudoPeriodic=off  Frequencies=[]  NoiseDistribution=none  NoiseParameters=[]  Unit=m  AffineConversion=off  FilteringAndDerivatives=provide  SimscapeFilterOrder=1  InputFilterTimeConstant=0.001  UdotUserProvided=0
  To Workspace : ToWorkspace  VariableName=EXVRefPress_inMpa  SampleTime=-1
  To Workspace1 : ToWorkspace  VariableName=EXVRefPress_outMpa  SampleTime=-1
  Transfer Fcn : TransferFcn  Denominator=[1 1]
  B : PMIOPort  Side=Left
  A : PMIOPort  Port=2  Side=Right
  wires:
  Max Valve Displacement [m]/1 -> Scope/1, Simulink-PS Converter/1
  [cmd_exv_heatpump] -> Transfer Fcn/1
  Transfer Fcn/1 -> Max Valve Displacement [m]/1
  PS-Simulink Converter/1 -> To Workspace/1
  PS-Simulink Converter1/1 -> To Workspace1/1
  connections:
  Heat Pump Expansion Valve/RConn1 -- "Pressure, Temperature & Internal Energy Sensor (2P)1"/LConn1 -- B/RConn1
  Heat Pump Expansion Valve/LConn1 -- "Pressure, Temperature & Internal Energy Sensor (2P)"/LConn1 -- A/RConn1
  Heat Pump Expansion Valve/LConn2 -- Simulink-PS Converter/RConn1
  PS-Simulink Converter/LConn1 -- "Pressure, Temperature & Internal Energy Sensor (2P)"/RConn1
  PS-Simulink Converter1/LConn1 -- "Pressure, Temperature & Internal Energy Sensor (2P)1"/RConn1

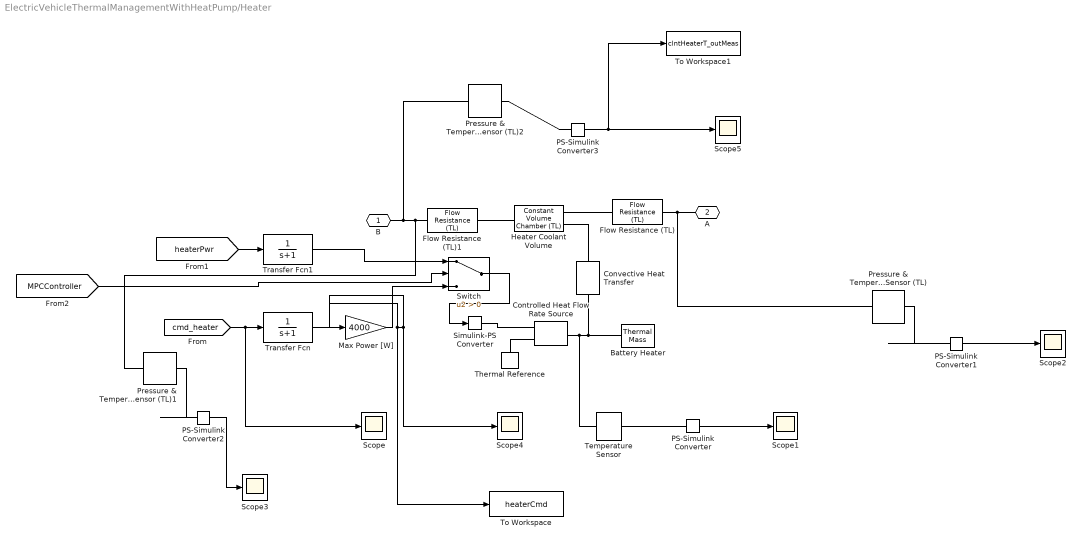
== system ElectricVehicleThermalManagementWithHeatPump/Heater ==
  Battery Heater : fl_lib/Thermal/Thermal Elements/Thermal Mass  mass_type=foundation.enum.constant_variable.constant  mass=2 kg  sp_heat=447 J/kg/K  mass_min=1e-6 kg  num_ports=foundation.enum.numPorts2.one  m_specify=off  m_priority=High  m=1 kg  m_nominal_specify=off  m_nominal_value=1  m_nominal_unit=kg  T_specify=on  T_priority=High  T=coolant_T_init degC  T_nominal_specify=off  T_nominal_value=1  T_nominal_unit=K  Q_specify=off  Q_priority=None  Q=0 W  Q_nominal_specify=off  Q_nominal_value=1  Q_nominal_unit=W
  Controlled Heat Flow Rate Source : fl_lib/Thermal/Thermal Sources/Controlled Heat Flow Rate Source
  Convective Heat Transfer : fl_lib/Thermal/Thermal Elements/Convective Heat Transfer  thermal_type=foundation.enum.constant_variable.constant  area=1 m^2  heat_tr_coeff=200 W/(m^2 * K)  min_heat_tr_coeff=1e-3 W/(K*m^2)  T_specify=off  T_priority=None  T=0 K  T_nominal_specify=off  T_nominal_value=1  T_nominal_unit=K  Q_specify=off  Q_priority=None  Q=0 W  Q_nominal_specify=off  Q_nominal_value=1  Q_nominal_unit=W
  Flow Resistance (TL) : fl_lib/Thermal Liquid/Elements/Flow Resistance (TL)  delta_p_nominal=2e-4 MPa  mdot_nominal=0.15 kg/s  area=pi * coolant_pipe_D^2 / 4 m^2  laminar_fraction=1e-3
  Flow Resistance (TL)1 : fl_lib/Thermal Liquid/Elements/Flow Resistance (TL)  delta_p_nominal=2e-4 MPa  mdot_nominal=0.15 kg/s  area=pi * coolant_pipe_D^2 / 4 m^2  laminar_fraction=1e-3
  Heater Coolant Volume : fl_lib/Thermal Liquid/Elements/Constant Volume Chamber (TL)  volume=0.001 m^3  num_ports=foundation.enum.num_ports.two  area_A=pi * coolant_pipe_D^2 / 4 m^2  area_B=pi * coolant_pipe_D^2 / 4 m^2  area_C=0.01 m^2  area_D=0.01 m^2  p_I_specify=on  p_I_priority=High  p_I=coolant_p_init MPa  p_I_nominal_specify=off  p_I_nominal_value=1  p_I_nominal_unit=MPa  T_I_specify=on  T_I_priority=High  T_I=coolant_T_init degC  T_I_nominal_specify=off  T_I_nominal_value=1  T_I_nominal_unit=K  u_I_specify=off  u_I_priority=None  u_I=83.90600000000001 kJ/kg  u_I_nominal_specify=off  u_I_nominal_value=1  u_I_nominal_unit=kJ/kg  rho_I_specify=off  rho_I_priority=None  rho_I=998.21 kg/m^3  rho_I_nominal_specify=off  rho_I_nominal_value=1  rho_I_nominal_unit=kg/m^3
      settings: InternalSimscapePortConfiguration="{\"Bottom\":[],\"Left\":[{\"id\":\"A\",\"label\":\"A\",\"type\":\"foundation.thermal_liquid.thermal_liquid\"},{\"id\":\"H\",\"label\":\"H\",\"type\":\"foundation.thermal.thermal\"}],\"Right\":[{\"id\":\"B\",\"label\":\"B\",\"type\":\"foundation.thermal_liquid.thermal_liquid\"}],\"Top\":[]}"
  Max Power [W] : Gain  Gain=4000
  PS-Simulink Converter{,1..3} (4 alike) : nesl_utility/PS-Simulink Converter  PhysicalDomain=network_engine_domain  SubClassName=ps_output  LeftPortType=input  RightPortType=output  PseudoPeriodic=off  Frequencies=[]  VectorFormat=inherit  Unit=inherit  AffineConversion=off
  Pressure & Temperature Sensor (TL) : fl_lib/Thermal Liquid/Sensors/Pressure & Temperature Sensor (TL)  reference=foundation.enum.MeasurementReference.absolute  pressure=false  pressure_spec=foundation.enum.PressureMeasementSpec.Absolute  temperature=true
      settings: InternalSimscapePortConfiguration="{\"Bottom\":[{\"id\":\"T\",\"label\":\"T\",\"type\":\"output\"}],\"Left\":[{\"id\":\"A\",\"label\":\"A\",\"type\":\"foundation.thermal_liquid.thermal_liquid\"}],\"Right\":[],\"Top\":[]}"
  Pressure & Temperature Sensor (TL)1 : fl_lib/Thermal Liquid/Sensors/Pressure & Temperature Sensor (TL)  reference=foundation.enum.MeasurementReference.absolute  pressure=false  pressure_spec=foundation.enum.PressureMeasementSpec.Absolute  temperature=true
      settings: InternalSimscapePortConfiguration="{\"Bottom\":[{\"id\":\"T\",\"label\":\"T\",\"type\":\"output\"}],\"Left\":[{\"id\":\"A\",\"label\":\"A\",\"type\":\"foundation.thermal_liquid.thermal_liquid\"}],\"Right\":[],\"Top\":[]}"
  Pressure & Temperature Sensor (TL)2 : fl_lib/Thermal Liquid/Sensors/Pressure & Temperature Sensor (TL)  reference=foundation.enum.MeasurementReference.absolute  pressure=false  pressure_spec=foundation.enum.PressureMeasementSpec.Absolute  temperature=true
      settings: InternalSimscapePortConfiguration="{\"Bottom\":[{\"id\":\"T\",\"label\":\"T\",\"type\":\"output\"}],\"Left\":[{\"id\":\"A\",\"label\":\"A\",\"type\":\"foundation.thermal_liquid.thermal_liquid\"}],\"Right\":[],\"Top\":[]}"
  Scope{,1..5} (6 alike) : Scope
  Simulink-PS Converter : nesl_utility/Simulink-PS Converter  PhysicalDomain=network_engine_domain  SubClassName=ps_input  LeftPortType=input  RightPortType=output  PseudoPeriodic=off  Frequencies=[]  NoiseDistribution=none  NoiseParameters=[]  Unit=1  AffineConversion=off  FilteringAndDerivatives=provide  SimscapeFilterOrder=1  InputFilterTimeConstant=0.001  UdotUserProvided=0
  Switch : Switch  Criteria=u2 > Threshold  SaturateOnIntegerOverflow=off  InputSameDT=off
  Temperature Sensor : fl_lib/Thermal/Thermal Sensors/Temperature Sensor  temperature_measure=foundation.enum.MeasurementReference.absolute
      settings: InternalSimscapePortConfiguration="{\"Bottom\":[],\"Left\":[{\"id\":\"A\",\"label\":\"A\",\"type\":\"foundation.thermal.thermal\"}],\"Right\":[{\"id\":\"T\",\"label\":\"T\",\"type\":\"output\"}],\"Top\":[]}"
  Thermal Reference : fl_lib/Thermal/Thermal Elements/Thermal Reference
  To Workspace : ToWorkspace  VariableName=heaterCmd  SampleTime=-1
  To Workspace1 : ToWorkspace  VariableName=clntHeaterT_outMeas  SampleTime=-1
  Transfer Fcn : TransferFcn  Denominator=[1 1]
  Transfer Fcn1 : TransferFcn  Denominator=[1 1]
  B : PMIOPort  Side=Left
  A : PMIOPort  Port=2  Side=Right
  wires:
  [cmd_heater] -> Scope/1, Transfer Fcn/1
  Transfer Fcn/1 -> To Workspace/1, Scope4/1, Max Power [W]/1
  PS-Simulink Converter/1 -> Scope1/1
  PS-Simulink Converter1/1 -> Scope2/1
  PS-Simulink Converter2/1 -> Scope3/1
  PS-Simulink Converter3/1 -> To Workspace1/1, Scope5/1
  [heaterPwr] -> Transfer Fcn1/1
  Max Power [W]/1 -> Switch/3
  Transfer Fcn1/1 -> Switch/1
  [MPCController] -> Switch/2
  Switch/1 -> Simulink-PS Converter/1
  connections:
  Battery Heater/LConn1 -- Temperature Sensor/LConn1 -- Controlled Heat Flow Rate Source/LConn1 -- Convective Heat Transfer/LConn1
  Convective Heat Transfer/RConn1 -- Heater Coolant Volume/LConn2
  Flow Resistance (TL)/LConn1 -- Pressure & Temperature Sensor (TL)/LConn1 -- A/RConn1
  Flow Resistance (TL)1/RConn1 -- Pressure & Temperature Sensor (TL)1/LConn1 -- Pressure & Temperature Sensor (TL)2/LConn1 -- B/RConn1
  Flow Resistance (TL)1/LConn1 -- Heater Coolant Volume/RConn1
  Flow Resistance (TL)/RConn1 -- Heater Coolant Volume/LConn1
  Thermal Reference/LConn1 -- Controlled Heat Flow Rate Source/RConn2
  Temperature Sensor/RConn1 -- PS-Simulink Converter/LConn1
  PS-Simulink Converter1/LConn1 -- Pressure & Temperature Sensor (TL)/RConn1
  PS-Simulink Converter2/LConn1 -- Pressure & Temperature Sensor (TL)1/RConn1
  PS-Simulink Converter3/LConn1 -- Pressure & Temperature Sensor (TL)2/RConn1
  Simulink-PS Converter/RConn1 -- Controlled Heat Flow Rate Source/RConn1

== system ElectricVehicleThermalManagementWithHeatPump/Inner Condenser ==
  Flow Rate Sensor (MA) : fl_lib/Moist Air/Sensors/Flow Rate Sensor (MA)  mass_flow_measure=true  volumetric_flow_measure=false  volumetric_flow_conditions=foundation.enum.volumetric_flow_conditions.actual  p_std=0.101325 MPa  T_std=20 degC  RH_std=0.65  energy_flow_measure=true  vapor_flow_measure=false  gas_flow_measure=false  droplets_flow_measure=false
      settings: InternalSimscapePortConfiguration="{\"Bottom\":[{\"id\":\"PHI\",\"label\":\"φ\",\"type\":\"output\"}],\"Left\":[{\"id\":\"A\",\"label\":\"A\",\"type\":\"foundation.moist_air.moist_air\"}],\"Right\":[{\"id\":\"B\",\"label\":\"B\",\"type\":\"foundation.moist_air.moist_air\"},{\"id\":\"M\",\"label\":\"M\",\"type\":\"output\"}],\"Top\":[]}"
  Inner Condenser : SimscapeFluids_lib/Heat Exchangers/Two-Phase Fluid - Moist Air/Condenser Evaporator (2P-MA)  flow_arrangement=fluids.heat_exchangers.enum.FlowArrangement2PMA.Cross  cross_flow_arrangement=fluids.heat_exchangers.enum.CrossFlowArrangement2PMA.UnmixedUnmixed  R_wall=inner_cond_wall_thickness / inner_cond_air_area_primary / inner_cond_wall_conductivity K/kW  area_A1=pi * refrigerant_pipe_D^2 / 4 m^2  area_B1=pi * refrigerant_pipe_D^2 / 4 m^2  area_A2=cabin_duct_area m^2  area_B2=cabin_duct_area m^2  tube_num_2P=inner_cond_N_tubes  tube_length_2P=inner_cond_L m  tube_cross_section_2P=fluids.heat_exchangers.enum.TubeCrossSection.Rectangular  tube_diameter_2P=0.05 m  tube_width_2P=inner_cond_W m  tube_height_2P=inner_cond_tube_H m  tube_inner_diameter_2P=0.05 m  tube_outer_diameter_2P=0.1 m  tube_flow_area_2P=0.002 m^2  tube_wetted_perimeter_2P=0.15 m  tube_heat_perimeter_2P=0.15 m  tube_pressure_loss_spec_2P=fluids.heat_exchangers.enum.TubePressureLossSpec2P.Haaland  tube_loss_coeff_2P=10  tube_local_pressure_loss_spec_2P=fluids.heat_exchangers.enum.LocalLossSpec.AggregateLength  tube_length_add_2P=inner_cond_tube_Leq m  tube_local_loss_coefficient_2P=0.1  tube_roughness_pressure_2P=15e-6 m  tube_Re_lam_pressure_2P=2000  tube_Re_tur_pressure_2P=4000  tube_shape_factor_generic_2P=64  tube_heat_coeff_spec_2P=fluids.heat_exchangers.enum.TubeHeatCoeffSpec2P.GneilinskiCavalliniZecchin  tube_colburn_coeff_liq_2P=[.023, .8, .33]  tube_colburn_coeff_mix_2P=[.05, .8, .33]  tube_colburn_coeff_vap_2P=[.023, .8, .33]  tube_roughness_heat_2P=15e-6 m  tube_Re_lam_heat_2P=2000  tube_Re_tur_heat_2P=4000  tube_Nu_lam_generic_2P=3.66  fouling_factor_2P=0.1 K*m^2/kW  fin_area_2P=inner_cond_tube_area_webs m^2  fin_efficiency_2P=0.6  energy_spec_2P=foundation.enum.energy_spec.void_fraction  p_init_2P=refrigerant_p_init MPa  T_init_2P=293.15 K  x_init_2P=0.5  alpha_init_2P=refrigerant_alpha_init  h_init_2P=1500 kJ/kg  u_init_2P=1500 kJ/kg  flow_geometry_MA=fluids.heat_exchangers.enum.FlowGeometryMA.Generic  tube_num_MA=25  tube_length_MA=1 m  tube_cross_section_MA=fluids.heat_exchangers.enum.TubeCrossSection.Circular  tube_diameter_MA=0.05 m  tube_width_MA=0.05 m  tube_height_MA=0.05 m  tube_inner_diameter_MA=0.05 m  tube_outer_diameter_MA=0.1 m  tube_flow_area_MA=0.002 m^2  tube_wetted_perimeter_MA=0.15 m  tube_heat_perimeter_MA=0.15 m  tube_pressure_loss_spec_MA=fluids.heat_exchangers.enum.TubePressureLossSpec.Haaland  tube_loss_coeff_MA=10  tube_local_pressure_loss_spec_MA=fluids.heat_exchangers.enum.LocalLossSpec.AggregateLength  tube_length_add_MA=0.1 m  tube_local_loss_coefficient_MA=0.1  tube_roughness_pressure_MA=15e-6 m  tube_Re_lam_pressure_MA=2000  tube_Re_tur_pressure_MA=4000  tube_shape_factor_generic_MA=64  tube_heat_coeff_spec_MA=fluids.heat_exchangers.enum.TubeHeatCoeffSpec.Gneilinski  tube_colburn_coeff_MA=[.023, .8, .33]  tube_roughness_heat_MA=15e-6 m  tube_Re_lam_heat_MA=2000  tube_Re_tur_heat_MA=4000  tube_Nu_lam_generic_MA=3.66  bank_arrangement_MA=fluids.heat_exchangers.enum.BankArrangement.Inline  bank_num_rows_MA=5  bank_tubes_per_row_MA=5  bank_width_MA=1 m  bank_tube_diameter_MA=0.05 m  bank_longitudinal_pitch_MA=0.15 m  bank_transverse_pitch_MA=0.15 m  bank_pressure_loss_spec_MA=fluids.heat_exchangers.enum.BankPressureLossSpec.Martin  bank_euler_MA=10  bank_heat_coeff_spec_MA=fluids.heat_exchangers.enum.BankHeatCoeffSpec.Martin  bank_colburn_coeff_MA=[.27, .63, .36]  generic_flow_area_MA=inner_cond_air_area_flow m^2  generic_heat_area_MA=inner_cond_air_area_primary m^2  generic_volume_MA=inner_cond_air_area_flow * inner_cond_W m^3  generic_loss_coeff_MA=10  generic_colburn_coeff_MA=[.023, .8, .33]  fouling_factor_MA=0.1 K*m^2/kW  fin_area_MA=inner_cond_air_area_fins m^2  fin_efficiency_MA=0.7  p_init_MA=cabin_p_init MPa  T_init_MA=cabin_T_init degC  humidity_spec_MA=foundation.enum.HumiditySpec.RelativeHumidity  RH_init_MA=cabin_RH_init  x_w_init_MA=0.01  y_w_init_MA=0.01  HR_init_MA=0.01  Tw_init_MA=287 K  trace_gas_spec_MA=foundation.enum.trace_gas_spec.mole_fraction  x_g_init_MA=0.001  y_g_init_MA=cabin_CO2_init  r_d_init_MA=0  RH_ws_MA=1  time_constant_cond_MA=1e-3 s  time_constant_evap_MA=1e-3 s  fraction_entrained_MA=1
      settings: InternalSimscapePortConfiguration="{\"Bottom\":[],\"Left\":[{\"id\":\"A1\",\"label\":\"A1\",\"type\":\"foundation.two_phase_fluid.two_phase_fluid\"},{\"id\":\"Z\",\"label\":\"Z\",\"type\":\"output\"},{\"id\":\"B1\",\"label\":\"B1\",\"type\":\"foundation.two_phase_fluid.two_phase_fluid\"}],\"Right\":[{\"id\":\"A2\",\"label\":\"A2\",\"type\":\"foundation.moist_air.moist_air\"},{\"id\":\"W\",\"label\":\"W\",\"type\":\"output\"},{\"id\":\"B2\",\"label\":\"B2\",\"type\":\"foundation.moist_air.moist_air\"}],\"Top\":[]}"
  PS-Simulink Converter : nesl_utility/PS-Simulink Converter  PhysicalDomain=network_engine_domain  SubClassName=ps_output  LeftPortType=input  RightPortType=output  PseudoPeriodic=off  Frequencies=[]  VectorFormat=inherit  Unit=inherit  AffineConversion=off
  PS-Simulink Converter1 : nesl_utility/PS-Simulink Converter  PhysicalDomain=network_engine_domain  SubClassName=ps_output  LeftPortType=input  RightPortType=output  PseudoPeriodic=off  Frequencies=[]  VectorFormat=inherit  Unit=inherit  AffineConversion=off
  PS-Simulink Converter2 : nesl_utility/PS-Simulink Converter  PhysicalDomain=network_engine_domain  SubClassName=ps_output  LeftPortType=input  RightPortType=output  PseudoPeriodic=off  Frequencies=[]  VectorFormat=inherit  Unit=inherit  AffineConversion=off
  Pressure & Temperature Sensor (MA) : fl_lib/Moist Air/Sensors/Pressure & Temperature Sensor (MA)  reference=foundation.enum.MeasurementReference.absolute  pressure=false  pressure_spec=foundation.enum.PressureMeasementSpec.Absolute  temperature=true
      settings: InternalSimscapePortConfiguration="{\"Bottom\":[{\"id\":\"T\",\"label\":\"T\",\"type\":\"output\"}],\"Left\":[{\"id\":\"A\",\"label\":\"A\",\"type\":\"foundation.moist_air.moist_air\"}],\"Right\":[],\"Top\":[]}"
  Pressure & Temperature Sensor (MA)1 : fl_lib/Moist Air/Sensors/Pressure & Temperature Sensor (MA)  reference=foundation.enum.MeasurementReference.absolute  pressure=false  pressure_spec=foundation.enum.PressureMeasementSpec.Absolute  temperature=true
      settings: InternalSimscapePortConfiguration="{\"Bottom\":[{\"id\":\"T\",\"label\":\"T\",\"type\":\"output\"}],\"Left\":[{\"id\":\"A\",\"label\":\"A\",\"type\":\"foundation.moist_air.moist_air\"}],\"Right\":[],\"Top\":[]}"
  SR1 : Subsystem
  SR2 : Subsystem
  Scope : Scope
  Scope1 : Scope
  Scope2 : Scope
  To Workspace : ToWorkspace  VariableName=innerCondAirTemp_inK  SampleTime=-1
  To Workspace1 : ToWorkspace  VariableName=innerCondAirTemp_outK  SampleTime=-1
  To Workspace2 : ToWorkspace  VariableName=airMassFlowRateCabin_in  SampleTime=-1
  C : PMIOPort  Side=Left
  B : PMIOPort  Port=2  Side=Left
  D : PMIOPort  Port=3  Side=Right
  A : PMIOPort  Port=4  Side=Right
  wires:
  PS-Simulink Converter/1 -> Scope2/1, To Workspace/1
  PS-Simulink Converter1/1 -> Scope1/1, To Workspace1/1
  PS-Simulink Converter2/1 -> Scope/1, To Workspace2/1
  connections:
  SR2/RConn1 -- B/RConn1
  SR1/LConn1 -- A/RConn1
  Inner Condenser/LConn1 -- SR1/RConn1
  Inner Condenser/LConn3 -- SR2/LConn1
  Inner Condenser/RConn3 -- C/RConn1 -- Pressure & Temperature Sensor (MA)/LConn1
  Inner Condenser/RConn1 -- Flow Rate Sensor (MA)/LConn1 -- Pressure & Temperature Sensor (MA)1/LConn1
  PS-Simulink Converter/LConn1 -- Pressure & Temperature Sensor (MA)/RConn1
  PS-Simulink Converter1/LConn1 -- Pressure & Temperature Sensor (MA)1/RConn1
  PS-Simulink Converter2/LConn1 -- Flow Rate Sensor (MA)/RConn2
  Flow Rate Sensor (MA)/RConn1 -- D/RConn1
